simulink model "solar_pv_protected_c07_circuit"  (R2026b)
settings: Solver=VariableStepAuto
model workspace (MAT data in the model file):
  candidate_owner = 'pv_protection_integration_20261023_r01'
  solar_edit_metadata : object (value not decoded)
libraries: fl_lib x149, ee_lib x16, ltc4364demo_lib x3, batteryecm_lib x1, solarprotect_lib x1
(part 16 of 16)

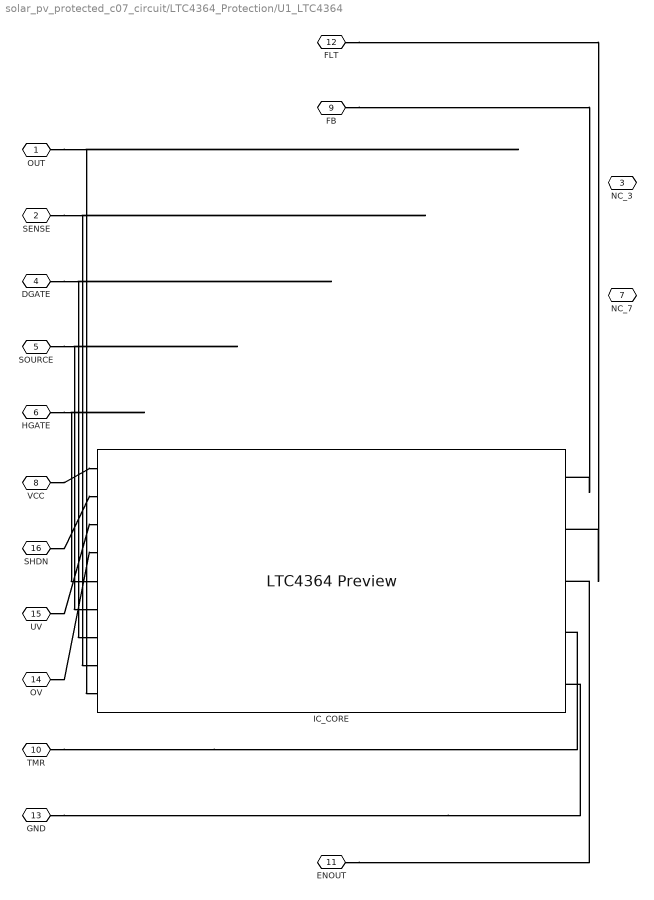
== system solar_pv_protected_c07_circuit/LTC4364_Protection/U1_LTC4364 ==
  IC_CORE : solarprotect_lib/LTC4364 Preview  Description=|  Vgate=12 V  Vref=1.25 V  VsenseLimit=0.05 V  VdiodeReg=0.03 V  ih_specify=off  ih_priority=None  ih=0 A  ih_nominal_specify=off  ih_nominal_value=1  ih_nominal_unit=A  iDG_specify=off  iDG_priority=None  iDG=0 A  iDG_nominal_specify=off  iDG_nominal_value=1  iDG_nominal_unit=A  ivcc_specify=off  ivcc_priority=None  ivcc=0 A  ivcc_nominal_specify=off  ivcc_nominal_value=1  ivcc_nominal_unit=A  ishdn_specify=off  ishdn_priority=None  ishdn=0 A  ishdn_nominal_specify=off  ishdn_nominal_value=1  ishdn_nominal_unit=A  iuv_specify=off  iuv_priority=None  iuv=0 A  iuv_nominal_specify=off  iuv_nominal_value=1  iuv_nominal_unit=A  iov_specify=off  iov_priority=None  iov=0 A  iov_nominal_specify=off  iov_nominal_value=1  iov_nominal_unit=A  ifb_specify=off  ifb_priority=None  ifb=0 A  ifb_nominal_specify=off  ifb_nominal_value=1  ifb_nominal_unit=A  itmr_specify=off  itmr_priority=None  itmr=0 A  itmr_nominal_specify=off  itmr_nominal_value=1  itmr_nominal_unit=A  isense_specify=off  isense_priority=None  isense=0 A  isense_nominal_specify=off  isense_nominal_value=1  isense_nominal_unit=A  iout_specify=off  iout_priority=None  iout=0 A  iout_nominal_specify=off  iout_nominal_value=1  iout_nominal_unit=A  iflt_specify=off  iflt_priority=None  iflt=0 A  iflt_nominal_specify=off  iflt_nominal_value=1  iflt_nominal_unit=A  ien_specify=off  ien_priority=None  ien=0 A  ien_nominal_specify=off  ien_nominal_value=1  ien_nominal_unit=A  latched_specify=off  latched_priority=None  latched=0  armed_specify=off  armed_priority=None  armed=0  uvReady_specify=off  uvReady_priority=None  uvReady=0
      | この回路での名前　　; LTC4364_Protection/U1_LTC4364/IC_CORE（内部モデル）
      | 部品名　　　　　　　; P_U1 / LTC4364IMS-1#PBFの内部表現
      | この回路での役割　　; 保護IC P_U1が電圧や電流の状態を見て、電流を通す・止める外付け素子を動かす働きを、モデル内部で近似する要素。
      | ここでの動き　　　　; プロジェクトで作成した機能近似を使う。メーカー提供の認証済みモデルではなく、実部品を追加したものでもない。
      | 
      | 【モデルの詳細・確認の範囲】
      | モデル内区分　　　　; P_U1 LTC4364の機能近似を実装するプロジェクト作成Simscapeコンポーネント。
      | 対応する実部品　　　; P_U1 / LTC4364IMS-1#PBF
      | モデルの範囲　　　　; 内部IC_COREにプロジェクト作成のLTC4364機能近似モデルを置く。メーカーの認証済みSimscapeモデルではない。限定試験の結果と実部品の高速過渡・SOA・熱の適合を区別する。
      | 説明の参照　　　　　; 上位部品ブロックのDescriptionに目的・接続・型番・未確認事項を記す。
      | 確認の範囲　　　　　; 説明整理のみ。実部品の全特性への同定や新たな動作試験を示さない。
      | 
      | 【この説明欄の略語・記号】
      | 用語1　　　　　　　 ; IC：Integrated Circuit（集積回路）。複数の電子素子と機能を小さな半導体チップに集積した部品。
      | 用語2　　　　　　　 ; SOA：Safe Operating Area（安全動作領域）。素子が扱える電圧・電流・継続時間・温度の組合せ。耐圧や最大電流を個別に満たすだけではSOAの成立にならない。
  OUT : PMIOPort  Description=|  Side=Left
      | 識別名　　　　　　　; OUT
      | 種別　　　　　　　　; Simscape Connection Port（階層境界の物理端子）
      | 所属部品　　　　　　; LTC4364_Protection/U1_LTC4364
      | 配置目的　　　　　　; 内部の電気ノードを、この外箱の外側の対応端子へ引き出す。
      | 対応端子　　　　　　; lconn:9
      | 接続ラベル　　　　　; BAT_PLUS
      | モデルの範囲　　　　; 実部品を1個追加する表現ではない。端子自体に増幅・遮断・測定機能を持たない。
      | 端子番号の注意　　　; Connection Portの番号は外箱内の対応番号であり、実パッケージのピン番号とは区別する。
      | 確認の範囲　　　　　; 実ポートと階層対応による静的接続の説明。電気特性の再現性は所属部品の説明を参照する。
  SENSE : PMIOPort  Description=|  Port=2  Side=Left
      | 識別名　　　　　　　; SENSE
      | 種別　　　　　　　　; Simscape Connection Port（階層境界の物理端子）
      | 所属部品　　　　　　; LTC4364_Protection/U1_LTC4364
      | 配置目的　　　　　　; 内部の電気ノードを、この外箱の外側の対応端子へ引き出す。
      | 対応端子　　　　　　; lconn:8
      | 接続ラベル　　　　　; ラベルなし。接続は実線と境界対応で定義する。
      | モデルの範囲　　　　; 実部品を1個追加する表現ではない。端子自体に増幅・遮断・測定機能を持たない。
      | 端子番号の注意　　　; Connection Portの番号は外箱内の対応番号であり、実パッケージのピン番号とは区別する。
      | 確認の範囲　　　　　; 実ポートと階層対応による静的接続の説明。電気特性の再現性は所属部品の説明を参照する。
  NC_3 : PMIOPort  Description=|  Port=3  Side=Left
      | この回路での名前　　; P_U1 / 3番端子
      | 端子機能　　　　　　; NC（No Connect：接続しない端子）
      | この回路での役割　　; MSOP-16の実物と端子番号を照合するための未接続端子。内部IC_COREにも外部回路にも接続しない。
      | メーカー根拠　　　　; https://www.analog.com/media/en/technical-documentation/data-sheets/ltc4364-1-4364-2.pdf
  DGATE : PMIOPort  Description=|  Port=4  Side=Left
      | 識別名　　　　　　　; DGATE
      | 種別　　　　　　　　; Simscape Connection Port（階層境界の物理端子）
      | 所属部品　　　　　　; LTC4364_Protection/U1_LTC4364
      | 配置目的　　　　　　; 内部の電気ノードを、この外箱の外側の対応端子へ引き出す。
      | 対応端子　　　　　　; lconn:7
      | 接続ラベル　　　　　; ラベルなし。接続は実線と境界対応で定義する。
      | モデルの範囲　　　　; 実部品を1個追加する表現ではない。端子自体に増幅・遮断・測定機能を持たない。
      | 端子番号の注意　　　; Connection Portの番号は外箱内の対応番号であり、実パッケージのピン番号とは区別する。
      | 確認の範囲　　　　　; 実ポートと階層対応による静的接続の説明。電気特性の再現性は所属部品の説明を参照する。
      | 
      | 【この説明欄の略語・記号】
      | 用語1　　　　　　　 ; PWM：Pulse Width Modulation（パルス幅変調）。周期に対するON時間の割合を変えて、スイッチの平均的な電力伝達を調整する方式。
      | 用語2　　　　　　　 ; MOSFET：Metal-Oxide-Semiconductor Field-Effect Transistor（金属・酸化膜・半導体構造の電界効果トランジスタ）。ゲートとソースの電圧でドレインとソースの導通を制御する素子。N-MOSはNチャネル型を表す。
      | 用語3　　　　　　　 ; HGATE/DGATE：LTC4364の二つの外付けMOSFETゲート駆動出力。HGATEは主に電圧・電流制限側のP_Q1、DGATEは理想ダイオード／逆流防止側のP_Q2を駆動する。主電力段の上下PWMとは別の仕組み。
  SOURCE : PMIOPort  Description=|  Port=5  Side=Left
      | 識別名　　　　　　　; SOURCE
      | 種別　　　　　　　　; Simscape Connection Port（階層境界の物理端子）
      | 所属部品　　　　　　; LTC4364_Protection/U1_LTC4364
      | 配置目的　　　　　　; 内部の電気ノードを、この外箱の外側の対応端子へ引き出す。
      | 対応端子　　　　　　; lconn:6
      | 接続ラベル　　　　　; ラベルなし。接続は実線と境界対応で定義する。
      | モデルの範囲　　　　; 実部品を1個追加する表現ではない。端子自体に増幅・遮断・測定機能を持たない。
      | 端子番号の注意　　　; Connection Portの番号は外箱内の対応番号であり、実パッケージのピン番号とは区別する。
      | 確認の範囲　　　　　; 実ポートと階層対応による静的接続の説明。電気特性の再現性は所属部品の説明を参照する。
  HGATE : PMIOPort  Description=|  Port=6  Side=Left
      | 識別名　　　　　　　; HGATE
      | 種別　　　　　　　　; Simscape Connection Port（階層境界の物理端子）
      | 所属部品　　　　　　; LTC4364_Protection/U1_LTC4364
      | 配置目的　　　　　　; 内部の電気ノードを、この外箱の外側の対応端子へ引き出す。
      | 対応端子　　　　　　; lconn:5
      | 接続ラベル　　　　　; ラベルなし。接続は実線と境界対応で定義する。
      | モデルの範囲　　　　; 実部品を1個追加する表現ではない。端子自体に増幅・遮断・測定機能を持たない。
      | 端子番号の注意　　　; Connection Portの番号は外箱内の対応番号であり、実パッケージのピン番号とは区別する。
      | 確認の範囲　　　　　; 実ポートと階層対応による静的接続の説明。電気特性の再現性は所属部品の説明を参照する。
      | 
      | 【この説明欄の略語・記号】
      | 用語1　　　　　　　 ; PWM：Pulse Width Modulation（パルス幅変調）。周期に対するON時間の割合を変えて、スイッチの平均的な電力伝達を調整する方式。
      | 用語2　　　　　　　 ; MOSFET：Metal-Oxide-Semiconductor Field-Effect Transistor（金属・酸化膜・半導体構造の電界効果トランジスタ）。ゲートとソースの電圧でドレインとソースの導通を制御する素子。N-MOSはNチャネル型を表す。
      | 用語3　　　　　　　 ; HGATE/DGATE：LTC4364の二つの外付けMOSFETゲート駆動出力。HGATEは主に電圧・電流制限側のP_Q1、DGATEは理想ダイオード／逆流防止側のP_Q2を駆動する。主電力段の上下PWMとは別の仕組み。
  NC_7 : PMIOPort  Description=|  Port=7  Side=Left
      | この回路での名前　　; P_U1 / 7番端子
      | 端子機能　　　　　　; NC（No Connect：接続しない端子）
      | この回路での役割　　; MSOP-16の実物と端子番号を照合するための未接続端子。内部IC_COREにも外部回路にも接続しない。
      | メーカー根拠　　　　; https://www.analog.com/media/en/technical-documentation/data-sheets/ltc4364-1-4364-2.pdf
  VCC : PMIOPort  Description=|  Port=8  Side=Left
      | 識別名　　　　　　　; VCC
      | 種別　　　　　　　　; Simscape Connection Port（階層境界の物理端子）
      | 所属部品　　　　　　; LTC4364_Protection/U1_LTC4364
      | 配置目的　　　　　　; 内部の電気ノードを、この外箱の外側の対応端子へ引き出す。
      | 対応端子　　　　　　; lconn:4
      | 接続ラベル　　　　　; ラベルなし。接続は実線と境界対応で定義する。
      | モデルの範囲　　　　; 実部品を1個追加する表現ではない。端子自体に増幅・遮断・測定機能を持たない。
      | 端子番号の注意　　　; Connection Portの番号は外箱内の対応番号であり、実パッケージのピン番号とは区別する。
      | 確認の範囲　　　　　; 実ポートと階層対応による静的接続の説明。電気特性の再現性は所属部品の説明を参照する。
      | 
      | 【この説明欄の略語・記号】
      | 用語1　　　　　　　 ; IC：Integrated Circuit（集積回路）。複数の電子素子と機能を小さな半導体チップに集積した部品。
      | 用語2　　　　　　　 ; MOSFET：Metal-Oxide-Semiconductor Field-Effect Transistor（金属・酸化膜・半導体構造の電界効果トランジスタ）。ゲートとソースの電圧でドレインとソースの導通を制御する素子。N-MOSはNチャネル型を表す。
      | 用語3　　　　　　　 ; GND：Ground（回路の基準電位・電流帰路）。この図の共通基準。保護接地や大地への接続を意味するとは限らない。
      | 用語4　　　　　　　 ; VCC/VDD/VEE/VS：ICの電源端子名。文字の歴史的な由来を現在の接続機能へ当てはめない。現回路のVEEはU8/U10では浮動基準SW、U9ではGND。各電圧・基準は端子と接続を参照する。
      | 用語5　　　　　　　 ; SW：Switching Node（スイッチング点）。主電力段の上下MOSFETとL1がつながる、電圧が高速に切り替わる点。GNDとは別電位。
  FB : PMIOPort  Description=|  Port=9  Side=Right
      | 識別名　　　　　　　; FB
      | 種別　　　　　　　　; Simscape Connection Port（階層境界の物理端子）
      | 所属部品　　　　　　; LTC4364_Protection/U1_LTC4364
      | 配置目的　　　　　　; 内部の電気ノードを、この外箱の外側の対応端子へ引き出す。
      | 対応端子　　　　　　; rconn:1
      | 接続ラベル　　　　　; ラベルなし。接続は実線と境界対応で定義する。
      | モデルの範囲　　　　; 実部品を1個追加する表現ではない。端子自体に増幅・遮断・測定機能を持たない。
      | 端子番号の注意　　　; Connection Portの番号は外箱内の対応番号であり、実パッケージのピン番号とは区別する。
      | 確認の範囲　　　　　; 実ポートと階層対応による静的接続の説明。電気特性の再現性は所属部品の説明を参照する。
      | 
      | 【この説明欄の略語・記号】
      | 用語1　　　　　　　 ; FB：Feedback（帰還）。出力などを検出して内部制御へ戻すための信号・端子。
  TMR : PMIOPort  Description=|  Port=10  Side=Right
      | 識別名　　　　　　　; TMR
      | 種別　　　　　　　　; Simscape Connection Port（階層境界の物理端子）
      | 所属部品　　　　　　; LTC4364_Protection/U1_LTC4364
      | 配置目的　　　　　　; 内部の電気ノードを、この外箱の外側の対応端子へ引き出す。
      | 対応端子　　　　　　; rconn:5
      | 接続ラベル　　　　　; ラベルなし。接続は実線と境界対応で定義する。
      | モデルの範囲　　　　; 実部品を1個追加する表現ではない。端子自体に増幅・遮断・測定機能を持たない。
      | 端子番号の注意　　　; Connection Portの番号は外箱内の対応番号であり、実パッケージのピン番号とは区別する。
      | 確認の範囲　　　　　; 実ポートと階層対応による静的接続の説明。電気特性の再現性は所属部品の説明を参照する。
      | 
      | 【この説明欄の略語・記号】
      | 用語1　　　　　　　 ; TMR：Timer（時間設定端子）。LTC4364では外付けコンデンサにより故障継続時間の判定などに関係する時間を設定する。
  ENOUT : PMIOPort  Description=|  Port=11  Side=Right
      | 識別名　　　　　　　; ENOUT
      | 種別　　　　　　　　; Simscape Connection Port（階層境界の物理端子）
      | 所属部品　　　　　　; LTC4364_Protection/U1_LTC4364
      | 配置目的　　　　　　; 内部の電気ノードを、この外箱の外側の対応端子へ引き出す。
      | 対応端子　　　　　　; rconn:2
      | 接続ラベル　　　　　; ラベルなし。接続は実線と境界対応で定義する。
      | モデルの範囲　　　　; 実部品を1個追加する表現ではない。端子自体に増幅・遮断・測定機能を持たない。
      | 端子番号の注意　　　; Connection Portの番号は外箱内の対応番号であり、実パッケージのピン番号とは区別する。
      | 確認の範囲　　　　　; 実ポートと階層対応による静的接続の説明。電気特性の再現性は所属部品の説明を参照する。
      | 
      | 【この説明欄の略語・記号】
      | 用語1　　　　　　　 ; SHDN：Shutdown（停止制御端子）。LTC4364ではLowで停止を指示する。Highは動作許可であり、保護判定を無効にするものではない。
      | 用語2　　　　　　　 ; ENOUT：Enable Output（動作許可状態の出力）。LTC4364の下流回路向け許可出力。SHDNへの外部停止指示とは方向が逆の別端子。
  FLT : PMIOPort  Description=|  Port=12  Side=Right
      | 識別名　　　　　　　; FLT
      | 種別　　　　　　　　; Simscape Connection Port（階層境界の物理端子）
      | 所属部品　　　　　　; LTC4364_Protection/U1_LTC4364
      | 配置目的　　　　　　; 内部の電気ノードを、この外箱の外側の対応端子へ引き出す。
      | 対応端子　　　　　　; rconn:3
      | 接続ラベル　　　　　; PROTECTION_FLT_N
      | モデルの範囲　　　　; 実部品を1個追加する表現ではない。端子自体に増幅・遮断・測定機能を持たない。
      | 端子番号の注意　　　; Connection Portの番号は外箱内の対応番号であり、実パッケージのピン番号とは区別する。
      | 確認の範囲　　　　　; 実ポートと階層対応による静的接続の説明。電気特性の再現性は所属部品の説明を参照する。
      | 
      | 【この説明欄の略語・記号】
      | 用語1　　　　　　　 ; FLT：Fault（故障状態通知）。LTC4364の故障警告出力。全種類の異常や逆流を一律に通知する信号という意味ではない。
  GND : PMIOPort  Description=|  Port=13  Side=Right
      | 識別名　　　　　　　; GND
      | 種別　　　　　　　　; Simscape Connection Port（階層境界の物理端子）
      | 所属部品　　　　　　; LTC4364_Protection/U1_LTC4364
      | 配置目的　　　　　　; 内部の電気ノードを、この外箱の外側の対応端子へ引き出す。
      | 対応端子　　　　　　; rconn:4
      | 接続ラベル　　　　　; GND、PROT_RETURN
      | モデルの範囲　　　　; 実部品を1個追加する表現ではない。端子自体に増幅・遮断・測定機能を持たない。
      | 端子番号の注意　　　; Connection Portの番号は外箱内の対応番号であり、実パッケージのピン番号とは区別する。
      | 確認の範囲　　　　　; 実ポートと階層対応による静的接続の説明。電気特性の再現性は所属部品の説明を参照する。
      | 
      | 【この説明欄の略語・記号】
      | 用語1　　　　　　　 ; GND：Ground（回路の基準電位・電流帰路）。この図の共通基準。保護接地や大地への接続を意味するとは限らない。
      | 用語2　　　　　　　 ; PROT_RETURN：保護回路の共通帰路。PROTはProtection（保護）、RETURNは帰路。プロトタイプの略ではなく、現回路では共通GNDへつながる。
  OV : PMIOPort  Description=|  Port=14  Side=Right
      | 識別名　　　　　　　; OV
      | 種別　　　　　　　　; Simscape Connection Port（階層境界の物理端子）
      | 所属部品　　　　　　; LTC4364_Protection/U1_LTC4364
      | 配置目的　　　　　　; 内部の電気ノードを、この外箱の外側の対応端子へ引き出す。
      | 対応端子　　　　　　; lconn:3
      | 接続ラベル　　　　　; ラベルなし。接続は実線と境界対応で定義する。
      | モデルの範囲　　　　; 実部品を1個追加する表現ではない。端子自体に増幅・遮断・測定機能を持たない。
      | 端子番号の注意　　　; Connection Portの番号は外箱内の対応番号であり、実パッケージのピン番号とは区別する。
      | 確認の範囲　　　　　; 実ポートと階層対応による静的接続の説明。電気特性の再現性は所属部品の説明を参照する。
      | 
      | 【この説明欄の略語・記号】
      | 用語1　　　　　　　 ; OV：Overvoltage（過電圧検出）。LTC4364の入力側過電圧判定。FBで行う出力電圧制限とは機能が異なる。
      | 用語2　　　　　　　 ; FB：Feedback（帰還）。出力などを検出して内部制御へ戻すための信号・端子。
  UV : PMIOPort  Description=|  Port=15  Side=Right
      | 識別名　　　　　　　; UV
      | 種別　　　　　　　　; Simscape Connection Port（階層境界の物理端子）
      | 所属部品　　　　　　; LTC4364_Protection/U1_LTC4364
      | 配置目的　　　　　　; 内部の電気ノードを、この外箱の外側の対応端子へ引き出す。
      | 対応端子　　　　　　; lconn:2
      | 接続ラベル　　　　　; ラベルなし。接続は実線と境界対応で定義する。
      | モデルの範囲　　　　; 実部品を1個追加する表現ではない。端子自体に増幅・遮断・測定機能を持たない。
      | 端子番号の注意　　　; Connection Portの番号は外箱内の対応番号であり、実パッケージのピン番号とは区別する。
      | 確認の範囲　　　　　; 実ポートと階層対応による静的接続の説明。電気特性の再現性は所属部品の説明を参照する。
      | 
      | 【この説明欄の略語・記号】
      | 用語1　　　　　　　 ; UV：Undervoltage（低電圧検出）。LTC4364の入力電圧が低い状態を判定する端子。
  SHDN : PMIOPort  Description=|  Port=16  Side=Right
      | 識別名　　　　　　　; SHDN
      | 種別　　　　　　　　; Simscape Connection Port（階層境界の物理端子）
      | 所属部品　　　　　　; LTC4364_Protection/U1_LTC4364
      | 配置目的　　　　　　; 内部の電気ノードを、この外箱の外側の対応端子へ引き出す。
      | 対応端子　　　　　　; lconn:1
      | 接続ラベル　　　　　; ラベルなし。接続は実線と境界対応で定義する。
      | モデルの範囲　　　　; 実部品を1個追加する表現ではない。端子自体に増幅・遮断・測定機能を持たない。
      | 端子番号の注意　　　; Connection Portの番号は外箱内の対応番号であり、実パッケージのピン番号とは区別する。
      | 確認の範囲　　　　　; 実ポートと階層対応による静的接続の説明。電気特性の再現性は所属部品の説明を参照する。
      | 
      | 【この説明欄の略語・記号】
      | 用語1　　　　　　　 ; SHDN：Shutdown（停止制御端子）。LTC4364ではLowで停止を指示する。Highは動作許可であり、保護判定を無効にするものではない。
  connections:
  TMR/RConn1 -- IC_CORE/RConn4
  GND/RConn1 -- IC_CORE/RConn5
  FLT/RConn1 -- IC_CORE/RConn2
  ENOUT/RConn1 -- IC_CORE/RConn3
  FB/RConn1 -- IC_CORE/RConn1
  OUT/RConn1 -- IC_CORE/LConn9
  SENSE/RConn1 -- IC_CORE/LConn8
  DGATE/RConn1 -- IC_CORE/LConn7
  SOURCE/RConn1 -- IC_CORE/LConn6
  HGATE/RConn1 -- IC_CORE/LConn5
  VCC/RConn1 -- IC_CORE/LConn1
  OV/RConn1 -- IC_CORE/LConn4
  UV/RConn1 -- IC_CORE/LConn3
  SHDN/RConn1 -- IC_CORE/LConn2

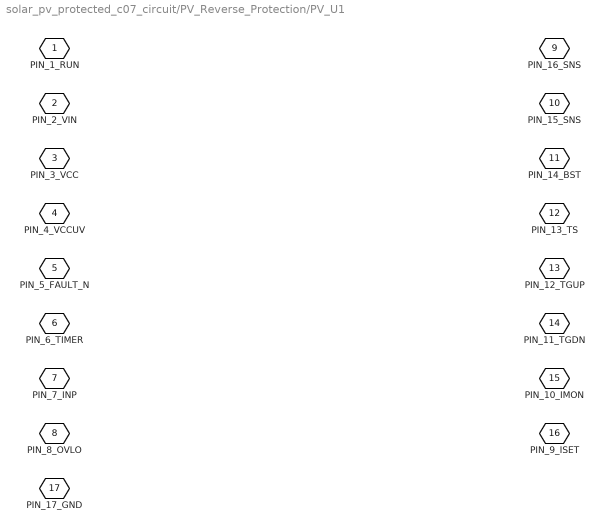
== system solar_pv_protected_c07_circuit/PV_Reverse_Protection/PV_U1 ==
  PIN_1_RUN : PMIOPort  Description=|  Side=Left  ConnectionType=Connection: foundation.electrical.electrical
      | 物理ピン番号        ; 1
      | 端子名              ; RUN
      | 接続先              ; PV_RUN_UV
      | この図の範囲        ; 実部品の端子番号に対応する接続口。この図面ではICの数値計算コアを除去している。対応する実行モデルの試験結果は別記録を参照。
  PIN_2_VIN : PMIOPort  Description=|  Port=2  Side=Left  ConnectionType=Connection: foundation.electrical.electrical
      | 物理ピン番号        ; 2
      | 端子名              ; VIN
      | 接続先              ; PV_IN
      | この図の範囲        ; 実部品の端子番号に対応する接続口。この図面ではICの数値計算コアを除去している。対応する実行モデルの試験結果は別記録を参照。
  PIN_3_VCC : PMIOPort  Description=|  Port=3  Side=Left  ConnectionType=Connection: foundation.electrical.electrical
      | 物理ピン番号        ; 3
      | 端子名              ; VCC
      | 接続先              ; PV_DRV_VCC
      | この図の範囲        ; 実部品の端子番号に対応する接続口。この図面ではICの数値計算コアを除去している。対応する実行モデルの試験結果は別記録を参照。
  PIN_4_VCCUV : PMIOPort  Description=|  Port=4  Side=Left  ConnectionType=Connection: foundation.electrical.electrical
      | 物理ピン番号        ; 4
      | 端子名              ; VCCUV
      | 接続先              ; PV_VCCUV
      | この図の範囲        ; 実部品の端子番号に対応する接続口。この図面ではICの数値計算コアを除去している。対応する実行モデルの試験結果は別記録を参照。
  PIN_5_FAULT_N : PMIOPort  Description=|  Port=5  Side=Left  ConnectionType=Connection: foundation.electrical.electrical
      | 物理ピン番号        ; 5
      | 端子名              ; FAULT_N
      | 接続先              ; OC_FAULT_N
      | この図の範囲        ; 実部品の端子番号に対応する接続口。この図面ではICの数値計算コアを除去している。対応する実行モデルの試験結果は別記録を参照。
  PIN_6_TIMER : PMIOPort  Description=|  Port=6  Side=Left  ConnectionType=Connection: foundation.electrical.electrical
      | 物理ピン番号        ; 6
      | 端子名              ; TIMER
      | 接続先              ; PV_TIMER
      | この図の範囲        ; 実部品の端子番号に対応する接続口。この図面ではICの数値計算コアを除去している。対応する実行モデルの試験結果は別記録を参照。
  PIN_7_INP : PMIOPort  Description=|  Port=7  Side=Left  ConnectionType=Connection: foundation.electrical.electrical
      | 物理ピン番号        ; 7
      | 端子名              ; INP
      | 接続先              ; PV_ALLOW
      | この図の範囲        ; 実部品の端子番号に対応する接続口。この図面ではICの数値計算コアを除去している。対応する実行モデルの試験結果は別記録を参照。
  PIN_8_OVLO : PMIOPort  Description=|  Port=8  Side=Left  ConnectionType=Connection: foundation.electrical.electrical
      | 物理ピン番号        ; 8
      | 端子名              ; OVLO
      | 接続先              ; PV_OV
      | この図の範囲        ; 実部品の端子番号に対応する接続口。この図面ではICの数値計算コアを除去している。対応する実行モデルの試験結果は別記録を参照。
  PIN_16_SNS : PMIOPort  Description=|  Port=9  Side=Right  ConnectionType=Connection: foundation.electrical.electrical
      | 物理ピン番号        ; 16
      | 端子名              ; SNS+
      | 接続先              ; PV_IN
      | この図の範囲        ; 実部品の端子番号に対応する接続口。この図面ではICの数値計算コアを除去している。対応する実行モデルの試験結果は別記録を参照。
  PIN_15_SNS : PMIOPort  Description=|  Port=10  Side=Right  ConnectionType=Connection: foundation.electrical.electrical
      | 物理ピン番号        ; 15
      | 端子名              ; SNS-
      | 接続先              ; PV_SNS_MINUS
      | この図の範囲        ; 実部品の端子番号に対応する接続口。この図面ではICの数値計算コアを除去している。対応する実行モデルの試験結果は別記録を参照。
  PIN_14_BST : PMIOPort  Description=|  Port=11  Side=Right  ConnectionType=Connection: foundation.electrical.electrical
      | 物理ピン番号        ; 14
      | 端子名              ; BST
      | 接続先              ; PV_BST
      | この図の範囲        ; 実部品の端子番号に対応する接続口。この図面ではICの数値計算コアを除去している。対応する実行モデルの試験結果は別記録を参照。
  PIN_13_TS : PMIOPort  Description=|  Port=12  Side=Right  ConnectionType=Connection: foundation.electrical.electrical
      | 物理ピン番号        ; 13
      | 端子名              ; TS
      | 接続先              ; PV_COMMON_SOURCE
      | この図の範囲        ; 実部品の端子番号に対応する接続口。この図面ではICの数値計算コアを除去している。対応する実行モデルの試験結果は別記録を参照。
  PIN_12_TGUP : PMIOPort  Description=|  Port=13  Side=Right  ConnectionType=Connection: foundation.electrical.electrical
      | 物理ピン番号        ; 12
      | 端子名              ; TGUP
      | 接続先              ; PV_GATE_UP
      | この図の範囲        ; 実部品の端子番号に対応する接続口。この図面ではICの数値計算コアを除去している。対応する実行モデルの試験結果は別記録を参照。
  PIN_11_TGDN : PMIOPort  Description=|  Port=14  Side=Right  ConnectionType=Connection: foundation.electrical.electrical
      | 物理ピン番号        ; 11
      | 端子名              ; TGDN
      | 接続先              ; PV_GATE
      | この図の範囲        ; 実部品の端子番号に対応する接続口。この図面ではICの数値計算コアを除去している。対応する実行モデルの試験結果は別記録を参照。
  PIN_10_IMON : PMIOPort  Description=|  Port=15  Side=Right  ConnectionType=Connection: foundation.electrical.electrical
      | 物理ピン番号        ; 10
      | 端子名              ; IMON
      | 接続先              ; NC（IMON未使用）
      | この図の範囲        ; 実部品の端子番号に対応する接続口。この図面ではICの数値計算コアを除去している。対応する実行モデルの試験結果は別記録を参照。
  PIN_9_ISET : PMIOPort  Description=|  Port=16  Side=Right  ConnectionType=Connection: foundation.electrical.electrical
      | 物理ピン番号        ; 9
      | 端子名              ; ISET
      | 接続先              ; GND
      | この図の範囲        ; 実部品の端子番号に対応する接続口。この図面ではICの数値計算コアを除去している。対応する実行モデルの試験結果は別記録を参照。
  PIN_17_GND : PMIOPort  Description=|  Port=17  Side=Left  ConnectionType=Connection: foundation.electrical.electrical
      | 物理ピン番号        ; 17
      | 端子名              ; GND
      | 接続先              ; GND
      | この図の範囲        ; 実部品の端子番号に対応する接続口。この図面ではICの数値計算コアを除去している。対応する実行モデルの試験結果は別記録を参照。

== system solar_pv_protected_c07_circuit/PV_Reverse_Protection/PV_U3 ==
  PIN_1_OUT : PMIOPort  Description=|  Side=Left  ConnectionType=Connection: foundation.electrical.electrical
      | 物理ピン番号        ; 1
      | 端子名              ; OUT
      | 接続先              ; REV_OK
      | この図の範囲        ; 実部品の端子番号に対応する接続口。この図面ではICの数値計算コアを除去している。対応する実行モデルの試験結果は別記録を参照。
  PIN_2_GND : PMIOPort  Description=|  Port=2  Side=Left  ConnectionType=Connection: foundation.electrical.electrical
      | 物理ピン番号        ; 2
      | 端子名              ; GND
      | 接続先              ; GND
      | この図の範囲        ; 実部品の端子番号に対応する接続口。この図面ではICの数値計算コアを除去している。対応する実行モデルの試験結果は別記録を参照。
  PIN_3_IN : PMIOPort  Description=|  Port=3  Side=Left  ConnectionType=Connection: foundation.electrical.electrical
      | 物理ピン番号        ; 3
      | 端子名              ; IN+
      | 接続先              ; IPV_OUT
      | この図の範囲        ; 実部品の端子番号に対応する接続口。この図面ではICの数値計算コアを除去している。対応する実行モデルの試験結果は別記録を参照。
  PIN_5_VCC : PMIOPort  Description=|  Port=4  Side=Right  ConnectionType=Connection: foundation.electrical.electrical
      | 物理ピン番号        ; 5
      | 端子名              ; VCC
      | 接続先              ; P3V3
      | この図の範囲        ; 実部品の端子番号に対応する接続口。この図面ではICの数値計算コアを除去している。対応する実行モデルの試験結果は別記録を参照。
  PIN_4_IN : PMIOPort  Description=|  Port=5  Side=Right  ConnectionType=Connection: foundation.electrical.electrical
      | 物理ピン番号        ; 4
      | 端子名              ; IN-
      | 接続先              ; V_REV
      | この図の範囲        ; 実部品の端子番号に対応する接続口。この図面ではICの数値計算コアを除去している。対応する実行モデルの試験結果は別記録を参照。

== system solar_pv_protected_c07_circuit/PV_Reverse_Protection/PV_U4 ==
  PIN_1_A : PMIOPort  Description=|  Side=Left  ConnectionType=Connection: foundation.electrical.electrical
      | 物理ピン番号        ; 1
      | 端子名              ; A
      | 接続先              ; REV_OK
      | この図の範囲        ; 実部品の端子番号に対応する接続口。この図面ではICの数値計算コアを除去している。対応する実行モデルの試験結果は別記録を参照。
  PIN_2_GND : PMIOPort  Description=|  Port=2  Side=Left  ConnectionType=Connection: foundation.electrical.electrical
      | 物理ピン番号        ; 2
      | 端子名              ; GND
      | 接続先              ; GND
      | この図の範囲        ; 実部品の端子番号に対応する接続口。この図面ではICの数値計算コアを除去している。対応する実行モデルの試験結果は別記録を参照。
  PIN_3_B : PMIOPort  Description=|  Port=3  Side=Left  ConnectionType=Connection: foundation.electrical.electrical
      | 物理ピン番号        ; 3
      | 端子名              ; B
      | 接続先              ; ANALOG_OK
      | この図の範囲        ; 実部品の端子番号に対応する接続口。この図面ではICの数値計算コアを除去している。対応する実行モデルの試験結果は別記録を参照。
  PIN_6_C : PMIOPort  Description=|  Port=4  Side=Right  ConnectionType=Connection: foundation.electrical.electrical
      | 物理ピン番号        ; 6
      | 端子名              ; C
      | 接続先              ; MCU_RUN
      | この図の範囲        ; 実部品の端子番号に対応する接続口。この図面ではICの数値計算コアを除去している。対応する実行モデルの試験結果は別記録を参照。
  PIN_5_VCC : PMIOPort  Description=|  Port=5  Side=Right  ConnectionType=Connection: foundation.electrical.electrical
      | 物理ピン番号        ; 5
      | 端子名              ; VCC
      | 接続先              ; P3V3
      | この図の範囲        ; 実部品の端子番号に対応する接続口。この図面ではICの数値計算コアを除去している。対応する実行モデルの試験結果は別記録を参照。
  PIN_4_Y : PMIOPort  Description=|  Port=6  Side=Right  ConnectionType=Connection: foundation.electrical.electrical
      | 物理ピン番号        ; 4
      | 端子名              ; Y
      | 接続先              ; ALLOW_CLEAR_N
      | この図の範囲        ; 実部品の端子番号に対応する接続口。この図面ではICの数値計算コアを除去している。対応する実行モデルの試験結果は別記録を参照。

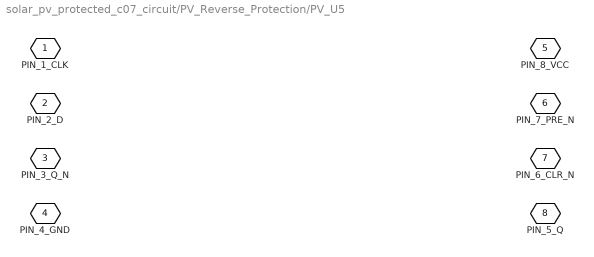
== system solar_pv_protected_c07_circuit/PV_Reverse_Protection/PV_U5 ==
  PIN_1_CLK : PMIOPort  Description=|  Side=Left  ConnectionType=Connection: foundation.electrical.electrical
      | 物理ピン番号        ; 1
      | 端子名              ; CLK
      | 接続先              ; MCU_REARM
      | この図の範囲        ; 実部品の端子番号に対応する接続口。この図面ではICの数値計算コアを除去している。対応する実行モデルの試験結果は別記録を参照。
  PIN_2_D : PMIOPort  Description=|  Port=2  Side=Left  ConnectionType=Connection: foundation.electrical.electrical
      | 物理ピン番号        ; 2
      | 端子名              ; D
      | 接続先              ; P3V3
      | この図の範囲        ; 実部品の端子番号に対応する接続口。この図面ではICの数値計算コアを除去している。対応する実行モデルの試験結果は別記録を参照。
  PIN_3_Q_N : PMIOPort  Description=|  Port=3  Side=Left  ConnectionType=Connection: foundation.electrical.electrical
      | 物理ピン番号        ; 3
      | 端子名              ; Q_N
      | 接続先              ; PV_STOPPED
      | この図の範囲        ; 実部品の端子番号に対応する接続口。この図面ではICの数値計算コアを除去している。対応する実行モデルの試験結果は別記録を参照。
  PIN_4_GND : PMIOPort  Description=|  Port=4  Side=Left  ConnectionType=Connection: foundation.electrical.electrical
      | 物理ピン番号        ; 4
      | 端子名              ; GND
      | 接続先              ; GND
      | この図の範囲        ; 実部品の端子番号に対応する接続口。この図面ではICの数値計算コアを除去している。対応する実行モデルの試験結果は別記録を参照。
  PIN_8_VCC : PMIOPort  Description=|  Port=5  Side=Right  ConnectionType=Connection: foundation.electrical.electrical
      | 物理ピン番号        ; 8
      | 端子名              ; VCC
      | 接続先              ; P3V3
      | この図の範囲        ; 実部品の端子番号に対応する接続口。この図面ではICの数値計算コアを除去している。対応する実行モデルの試験結果は別記録を参照。
  PIN_7_PRE_N : PMIOPort  Description=|  Port=6  Side=Right  ConnectionType=Connection: foundation.electrical.electrical
      | 物理ピン番号        ; 7
      | 端子名              ; PRE_N
      | 接続先              ; P3V3
      | この図の範囲        ; 実部品の端子番号に対応する接続口。この図面ではICの数値計算コアを除去している。対応する実行モデルの試験結果は別記録を参照。
  PIN_6_CLR_N : PMIOPort  Description=|  Port=7  Side=Right  ConnectionType=Connection: foundation.electrical.electrical
      | 物理ピン番号        ; 6
      | 端子名              ; CLR_N
      | 接続先              ; ALLOW_CLEAR_N
      | この図の範囲        ; 実部品の端子番号に対応する接続口。この図面ではICの数値計算コアを除去している。対応する実行モデルの試験結果は別記録を参照。
  PIN_5_Q : PMIOPort  Description=|  Port=8  Side=Right  ConnectionType=Connection: foundation.electrical.electrical
      | 物理ピン番号        ; 5
      | 端子名              ; Q
      | 接続先              ; PV_ALLOW
      | この図の範囲        ; 実部品の端子番号に対応する接続口。この図面ではICの数値計算コアを除去している。対応する実行モデルの試験結果は別記録を参照。

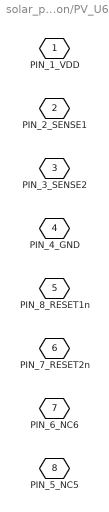
== system solar_pv_protected_c07_circuit/PV_Reverse_Protection/PV_U6 ==
  PIN_1_VDD : PMIOPort  Description=|  Side=Left  ConnectionType=Connection: foundation.electrical.electrical
      | 物理ピン番号        ; 1
      | 端子名              ; VDD
      | 接続先              ; P3V3
      | この図の範囲        ; 実部品の端子番号に対応する接続口。この図面ではICの数値計算コアを除去している。対応する実行モデルの試験結果は別記録を参照。
  PIN_2_SENSE1 : PMIOPort  Description=|  Port=2  Side=Left  ConnectionType=Connection: foundation.electrical.electrical
      | 物理ピン番号        ; 2
      | 端子名              ; SENSE1
      | 接続先              ; PV_SUP_3V3
      | この図の範囲        ; 実部品の端子番号に対応する接続口。この図面ではICの数値計算コアを除去している。対応する実行モデルの試験結果は別記録を参照。
  PIN_3_SENSE2 : PMIOPort  Description=|  Port=3  Side=Left  ConnectionType=Connection: foundation.electrical.electrical
      | 物理ピン番号        ; 3
      | 端子名              ; SENSE2
      | 接続先              ; PV_SUP_2V5
      | この図の範囲        ; 実部品の端子番号に対応する接続口。この図面ではICの数値計算コアを除去している。対応する実行モデルの試験結果は別記録を参照。
  PIN_4_GND : PMIOPort  Description=|  Port=4  Side=Left  ConnectionType=Connection: foundation.electrical.electrical
      | 物理ピン番号        ; 4
      | 端子名              ; GND
      | 接続先              ; GND
      | この図の範囲        ; 実部品の端子番号に対応する接続口。この図面ではICの数値計算コアを除去している。対応する実行モデルの試験結果は別記録を参照。
  PIN_8_RESET1n : PMIOPort  Description=|  Port=5  Side=Right  ConnectionType=Connection: foundation.electrical.electrical
      | 物理ピン番号        ; 8
      | 端子名              ; RESET1n
      | 接続先              ; ANALOG_OK
      | この図の範囲        ; 実部品の端子番号に対応する接続口。この図面ではICの数値計算コアを除去している。対応する実行モデルの試験結果は別記録を参照。
  PIN_7_RESET2n : PMIOPort  Description=|  Port=6  Side=Right  ConnectionType=Connection: foundation.electrical.electrical
      | 物理ピン番号        ; 7
      | 端子名              ; RESET2n
      | 接続先              ; ANALOG_OK
      | この図の範囲        ; 実部品の端子番号に対応する接続口。この図面ではICの数値計算コアを除去している。対応する実行モデルの試験結果は別記録を参照。
  PIN_6_NC6 : PMIOPort  Description=|  Port=7  Side=Right  ConnectionType=Connection: foundation.electrical.electrical
      | 物理ピン番号        ; 6
      | 端子名              ; NC6
      | 接続先              ; NC（未接続）
      | この図の範囲        ; 実部品の端子番号に対応する接続口。この図面ではICの数値計算コアを除去している。対応する実行モデルの試験結果は別記録を参照。
  PIN_5_NC5 : PMIOPort  Description=|  Port=8  Side=Right  ConnectionType=Connection: foundation.electrical.electrical
      | 物理ピン番号        ; 5
      | 端子名              ; NC5
      | 接続先              ; NC（未接続）
      | この図の範囲        ; 実部品の端子番号に対応する接続口。この図面ではICの数値計算コアを除去している。対応する実行モデルの試験結果は別記録を参照。

== system solar_pv_protected_c07_circuit/PV_Reverse_Protection/R27 ==
  Native_Shunt : fl_lib/Electrical/Electrical Elements/Resistor  Description=|  R=0.001 Ohm  i_specify=off  i_priority=None  i=0 A  i_nominal_specify=off  i_nominal_value=1  i_nominal_unit=A  v_specify=off  v_priority=None  v=0 V  v_nominal_specify=off  v_nominal_value=1  v_nominal_unit=V
      | この回路での名前　　; R27/Native_Shunt（内部モデル）
      | 部品名　　　　　　　; R27 / CSS4J-4026R-1L00Fの内部表現
      | この回路での役割　　; R27に電流が流れたときの小さな電圧差を、モデル内部で表す抵抗要素。実部品を追加したものではない。
      | ここでの動き　　　　; 外側の電流用端子と測定用端子を内部の抵抗につなぎ、電流と検出電圧の関係を表す。
      | 
      | 【モデルの詳細・確認の範囲】
      | モデル内区分　　　　; R27の電力端子間に置く標準抵抗。外側の測定端子と合わせてKelvin接続を表現する。
      | 対応する実部品　　　; R27 / CSS4J-4026R-1L00F
      | モデルの範囲　　　　; 4端子の接続を内部の標準抵抗へ割り当てた表現。Kelvin配線の抵抗・熱・磁気結合を実測同定したモデルではない。
      | 説明の参照　　　　　; 上位部品ブロックのDescriptionに目的・接続・型番・未確認事項を記す。
      | 確認の範囲　　　　　; 説明整理のみ。実部品の全特性への同定や新たな動作試験を示さない。
  Pin_001 : PMIOPort  Description=|  Side=Left  ConnectionType=Connection: foundation.electrical.electrical
      | 識別名　　　　　　　; Pin_001
      | 種別　　　　　　　　; Simscape Connection Port（階層境界の物理端子）
      | 所属部品　　　　　　; R27
      | 配置目的　　　　　　; 内部の電気ノードを、この外箱の外側の対応端子へ引き出す。
      | 対応端子　　　　　　; lconn:1／KP番 KP
      | 接続ラベル　　　　　; ラベルなし。接続は実線と境界対応で定義する。
      | モデルの範囲　　　　; 実部品を1個追加する表現ではない。端子自体に増幅・遮断・測定機能を持たない。
      | 端子番号の注意　　　; Connection Portの番号は外箱内の対応番号であり、実パッケージのピン番号とは区別する。
      | 確認の範囲　　　　　; 実ポートと階層対応による静的接続の説明。電気特性の再現性は所属部品の説明を参照する。
      | 
      | 従来の補足　　　　　; 以前のDescriptionを以下に保持する。
      | Physical R27 pin KP / KP
      | 
      | 【この説明欄の略語・記号】
      | 用語1　　　　　　　 ; IP/IM・KP/KM：4端子シャントの端子役割を区別する設計上の表記。IP/IMは主電流端子、KP/KMはKelvin（4端子測定）の検出端子。P/Mは正側・負側の区別であり、端子番号は採用部品の割当を参照する。
  Pin_002 : PMIOPort  Description=|  Port=2  Side=Left  ConnectionType=Connection: foundation.electrical.electrical
      | 識別名　　　　　　　; Pin_002
      | 種別　　　　　　　　; Simscape Connection Port（階層境界の物理端子）
      | 所属部品　　　　　　; R27
      | 配置目的　　　　　　; 内部の電気ノードを、この外箱の外側の対応端子へ引き出す。
      | 対応端子　　　　　　; lconn:2／KM番 KM
      | 接続ラベル　　　　　; ラベルなし。接続は実線と境界対応で定義する。
      | モデルの範囲　　　　; 実部品を1個追加する表現ではない。端子自体に増幅・遮断・測定機能を持たない。
      | 端子番号の注意　　　; Connection Portの番号は外箱内の対応番号であり、実パッケージのピン番号とは区別する。
      | 確認の範囲　　　　　; 実ポートと階層対応による静的接続の説明。電気特性の再現性は所属部品の説明を参照する。
      | 
      | 従来の補足　　　　　; 以前のDescriptionを以下に保持する。
      | Physical R27 pin KM / KM
      | 
      | 【この説明欄の略語・記号】
      | 用語1　　　　　　　 ; IP/IM・KP/KM：4端子シャントの端子役割を区別する設計上の表記。IP/IMは主電流端子、KP/KMはKelvin（4端子測定）の検出端子。P/Mは正側・負側の区別であり、端子番号は採用部品の割当を参照する。
  Pin_003 : PMIOPort  Description=|  Port=3  Side=Left  ConnectionType=Connection: foundation.electrical.electrical
      | 識別名　　　　　　　; Pin_003
      | 種別　　　　　　　　; Simscape Connection Port（階層境界の物理端子）
      | 所属部品　　　　　　; R27
      | 配置目的　　　　　　; 内部の電気ノードを、この外箱の外側の対応端子へ引き出す。
      | 対応端子　　　　　　; lconn:3／IP番 IP
      | 接続ラベル　　　　　; ラベルなし。接続は実線と境界対応で定義する。
      | モデルの範囲　　　　; 実部品を1個追加する表現ではない。端子自体に増幅・遮断・測定機能を持たない。
      | 端子番号の注意　　　; Connection Portの番号は外箱内の対応番号であり、実パッケージのピン番号とは区別する。
      | 確認の範囲　　　　　; 実ポートと階層対応による静的接続の説明。電気特性の再現性は所属部品の説明を参照する。
      | 
      | 従来の補足　　　　　; 以前のDescriptionを以下に保持する。
      | Physical R27 pin IP / IP
      | 
      | 【この説明欄の略語・記号】
      | 用語1　　　　　　　 ; IP/IM・KP/KM：4端子シャントの端子役割を区別する設計上の表記。IP/IMは主電流端子、KP/KMはKelvin（4端子測定）の検出端子。P/Mは正側・負側の区別であり、端子番号は採用部品の割当を参照する。
  Pin_004 : PMIOPort  Description=|  Port=4  Side=Right  ConnectionType=Connection: foundation.electrical.electrical
      | 識別名　　　　　　　; Pin_004
      | 種別　　　　　　　　; Simscape Connection Port（階層境界の物理端子）
      | 所属部品　　　　　　; R27
      | 配置目的　　　　　　; 内部の電気ノードを、この外箱の外側の対応端子へ引き出す。
      | 対応端子　　　　　　; rconn:1／IM番 IM
      | 接続ラベル　　　　　; ラベルなし。接続は実線と境界対応で定義する。
      | モデルの範囲　　　　; 実部品を1個追加する表現ではない。端子自体に増幅・遮断・測定機能を持たない。
      | 端子番号の注意　　　; Connection Portの番号は外箱内の対応番号であり、実パッケージのピン番号とは区別する。
      | 確認の範囲　　　　　; 実ポートと階層対応による静的接続の説明。電気特性の再現性は所属部品の説明を参照する。
      | 
      | 従来の補足　　　　　; 以前のDescriptionを以下に保持する。
      | Physical R27 pin IM / IM
      | 
      | 【この説明欄の略語・記号】
      | 用語1　　　　　　　 ; IP/IM・KP/KM：4端子シャントの端子役割を区別する設計上の表記。IP/IMは主電流端子、KP/KMはKelvin（4端子測定）の検出端子。P/Mは正側・負側の区別であり、端子番号は採用部品の割当を参照する。
  connections:
  Pin_002/RConn1 -- Pin_004/RConn1 -- Native_Shunt/RConn1
  Pin_001/RConn1 -- Pin_003/RConn1 -- Native_Shunt/LConn1

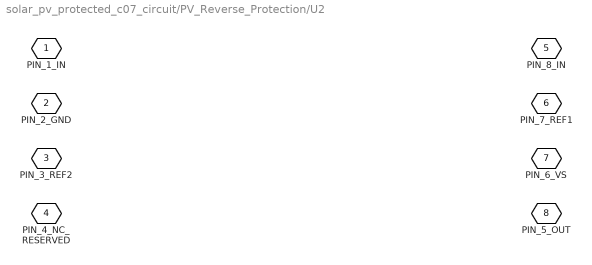
== system solar_pv_protected_c07_circuit/PV_Reverse_Protection/U2 ==
  PIN_1_IN : PMIOPort  Description=|  Side=Left  ConnectionType=Connection: foundation.electrical.electrical
      | 物理ピン番号        ; 1
      | 端子名              ; IN-
      | 接続先              ; PV_SENSED
      | この図の範囲        ; 実部品の端子番号に対応する接続口。この図面ではICの数値計算コアを除去している。対応する実行モデルの試験結果は別記録を参照。
  PIN_2_GND : PMIOPort  Description=|  Port=2  Side=Left  ConnectionType=Connection: foundation.electrical.electrical
      | 物理ピン番号        ; 2
      | 端子名              ; GND
      | 接続先              ; GND
      | この図の範囲        ; 実部品の端子番号に対応する接続口。この図面ではICの数値計算コアを除去している。対応する実行モデルの試験結果は別記録を参照。
  PIN_3_REF2 : PMIOPort  Description=|  Port=3  Side=Left  ConnectionType=Connection: foundation.electrical.electrical
      | 物理ピン番号        ; 3
      | 端子名              ; REF2
      | 接続先              ; GND
      | この図の範囲        ; 実部品の端子番号に対応する接続口。この図面ではICの数値計算コアを除去している。対応する実行モデルの試験結果は別記録を参照。
  PIN_4_NC_RESERVED : PMIOPort  Description=|  Port=4  Side=Left  ConnectionType=Connection: foundation.electrical.electrical
      | 物理ピン番号        ; 4
      | 端子名              ; NC_RESERVED
      | 接続先              ; GND
      | この図の範囲        ; 実部品の端子番号に対応する接続口。この図面ではICの数値計算コアを除去している。対応する実行モデルの試験結果は別記録を参照。
  PIN_8_IN : PMIOPort  Description=|  Port=5  Side=Right  ConnectionType=Connection: foundation.electrical.electrical
      | 物理ピン番号        ; 8
      | 端子名              ; IN+
      | 接続先              ; PV_IN
      | この図の範囲        ; 実部品の端子番号に対応する接続口。この図面ではICの数値計算コアを除去している。対応する実行モデルの試験結果は別記録を参照。
  PIN_7_REF1 : PMIOPort  Description=|  Port=6  Side=Right  ConnectionType=Connection: foundation.electrical.electrical
      | 物理ピン番号        ; 7
      | 端子名              ; REF1
      | 接続先              ; VREF2V5
      | この図の範囲        ; 実部品の端子番号に対応する接続口。この図面ではICの数値計算コアを除去している。対応する実行モデルの試験結果は別記録を参照。
  PIN_6_VS : PMIOPort  Description=|  Port=7  Side=Right  ConnectionType=Connection: foundation.electrical.electrical
      | 物理ピン番号        ; 6
      | 端子名              ; VS
      | 接続先              ; P3V3
      | この図の範囲        ; 実部品の端子番号に対応する接続口。この図面ではICの数値計算コアを除去している。対応する実行モデルの試験結果は別記録を参照。
  PIN_5_OUT : PMIOPort  Description=|  Port=8  Side=Right  ConnectionType=Connection: foundation.electrical.electrical
      | 物理ピン番号        ; 5
      | 端子名              ; OUT
      | 接続先              ; IPV_OUT
      | この図の範囲        ; 実部品の端子番号に対応する接続口。この図面ではICの数値計算コアを除去している。対応する実行モデルの試験結果は別記録を参照。
